simulink library "shapeBlocks"  (R2024a)
settings: Solver=VariableStepAuto  StartTime=0.0  StopTime=10.0  RelTol=1e-3
Description:
  | Blocks that compute the areas of shapes.
settings Model: ModifiedByFormat=matlabdomain  Creator=matlabdomain  LastModifiedBy=matlabdomain

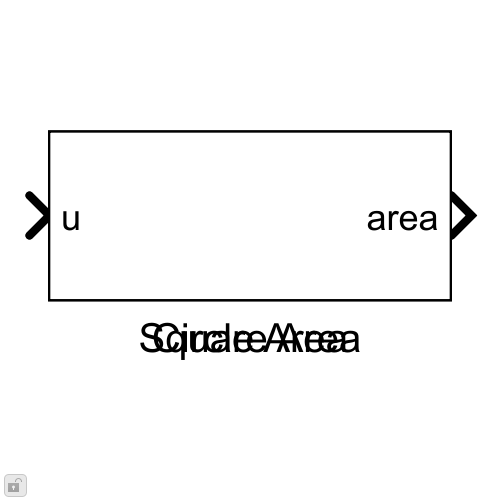
[thumbnail: Simulink's stored preview of the top-level diagram]
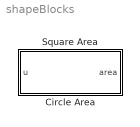
== system shapeBlocks ==
  Circle Area : Subsystem  mask(Shape area){scale=1, units=SI}
      mask prompts: scale "Scale factor"
      mask help: Area of a circle from its radius.
      mask TypeOptions units: SI | imperial
  Square Area : Subsystem  mask(Shape area){scale=1, units=SI}
      mask prompts: scale "Scale factor"
      mask help: Area of a square from its side.
      mask TypeOptions units: SI | imperial

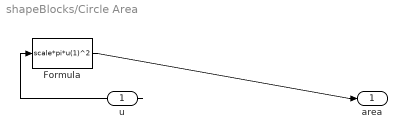
== system shapeBlocks/Circle Area ==
  u : Inport
  Formula : Fcn  Expr=scale*pi*u(1)^2
  area : Outport
  wires:
  u/1 -> Formula/1
  Formula/1 -> area/1

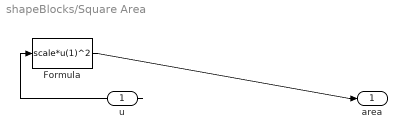
== system shapeBlocks/Square Area ==
  u : Inport
  Formula : Fcn  Expr=scale*u(1)^2
  area : Outport
  wires:
  u/1 -> Formula/1
  Formula/1 -> area/1
